simulink model "ASM_Traffic_MultiCore"  (R2026a)
settings: Solver=ode1  StartTime=SIM.tstart.v  StopTime=SIM.tend.v  FixedStep=SIM.StepSize.v
PostLoadFcn:
  | if any(exist('dsrtsu_mdlpostloadfcn', 'file') ~= 0), dsrtsu_mdlpostloadfcn('Execute', bdroot); end
  | try, asm_mdl_postloadfcn(bdroot, 'UpdateModel', 3600); catch, disp(lasterr); end,
InitFcn:
  | , if any(exist('rtifpga_mdlclblib', 'file') ~= 0), rtifpga_mdlclblib('Init', bdroot); end,
  | , if any(exist('dsmpb_private', 'file') ~= 0), dsmpb_private('dsmpb_mdlclblib', 'Init', bdroot); end,
model workspace (MAT data in the model file):
  asmReferencePath = [0 0.01 0.02 0.03 0.04 0.05 0.06 0.07 0.08 0.09 0.1 0.11 ... (350007 elements, 50001x7)]
  roadBounds : Simulink.Parameter (value not decoded)
  safetyAxes : Simulink.Parameter (value not decoded)
undefined symbols (not defined in the file): _to_, a0b2, ASM_BrakeHydraulics_DemoSystems, ASM_VehicleDynamics_DemoSystems, b98103fe8ad365046cd0, BrakeCircuit, controllerConfig, CPT, Crankshaft, DiscIntNeverNeededParam, dsmsi, FinalDriveAssembly, MDL, ModeSignals, mu, Pos_BrakePedal_Maneuver, rad, RefSignals, roadFamilyData, roadFamilyId, s_to_rpm, SIM, SoftECU, Suspension, Tire, Transmission
libraries: ASM_Traffic_lib x135, simulink x98, ASM_Utils_lib x77, ASM_VehicleDynamics_lib x70, ASM_Environment_lib x22, dsmpblib x20, dsmsilib x15, MDLD_Utils_lib x10, ASM_BrakeHydraulics_lib x3, sl_discontinuities x2
(part 22 of 65)

== system ASM_Traffic_MultiCore/Driver/Plant/UserInterface/ASMSignalBus_Plant ==
  In : Inport
  Terminator_1 : Terminator
  tag scope: ASMBUS_Driver_Plant=global
  wires:
  [ASMBUS_Driver_Plant] -> Terminator_1/1
  In/1 -> [ASMBUS_Driver_Plant]  "Plant"

== system ASM_Traffic_MultiCore/Driver/Plant/UserInterface/DISP_Plant ==
  Interface_In : Inport
  In : Inport  Port=2
  Angle_SteeringWheel[deg] : Subsystem
      mask Display: disp('')
  Bus Selector1 : BusSelector  OutputSignals=ReferenceVelocity.SpeedProfiler.a_x_Ref[m|s2],OutputSignals.Angle_SteeringWheel[deg],LateralController.PositionError.e_Lat[m]
  Bus Selector2 : BusSelector  OutputSignals=ReferenceVelocity.SpeedProfiler.v_x_Ref[km|h]
  Bus Selector3 : BusSelector  OutputSignals=OutputSignals.Pos_AccPedal[%],OutputSignals.Pos_BrakePedal[%],OutputSignals.Pos_ClutchPedal[%],OutputSignals.Gear[],OutputSignals.SelectorLever[-3T|-2P|-1R|0N|1D]
  Bus Selector4 : BusSelector  OutputSignals=ExternalModel.v_x_Vehicle[km|h]
  DRIVER : Scope  NumInputPorts=8
      settings: TimeSpan=5  ActiveDisplayYMinimum=-11.79033  ActiveDisplayYMaximum=105.56964  DataLoggingMaxPoints=20000  DataLoggingDecimation=10  DataLoggingVariableName=ScopeData2
  Err : Subsystem
  Gear[] : Subsystem
      mask Display: disp('')
  Mux : Mux  Inputs=2
  Mux1 : Mux  Inputs=3
  Mux2 : Mux  Inputs=2
  Pos_AccPedal[%] : Subsystem
      mask Display: disp('')
  Pos_BrakePedal[%] : Subsystem
      mask Display: disp('')
  Pos_ClutchPedal[%] : Subsystem
      mask Display: disp('')
  RelativeErr : Subsystem  mask{UpLim=100, LowLim=-100}
      mask prompts: UpLim "Upper Limit"; LowLim "Lower Limit"
  SelectorLever[-3T|-2P|-1R|0N|1D] : Subsystem
      mask Display: disp('')
  a_x_Vehicle_Ref[m|s2] : Subsystem
      mask Display: disp('')
  e_Lat[m] : Subsystem
      mask Display: disp('')
  v_Vehicle[km|h] : Subsystem
      mask Display: disp('')
  v_Vehicle_Ref[km|h] : Subsystem
      mask Display: disp('')
  wires:
  Angle_SteeringWheel[deg]/1(Out1) -> DRIVER/7  "Angle_SteeringWheel[deg]"
  e_Lat[m]/1(Out1) -> DRIVER/8  "e_Lat[m]"
  Bus Selector1/2 -> Angle_SteeringWheel[deg]/1(In1)  "<Angle_SteeringWheel[deg]>"
  Bus Selector1/3 -> e_Lat[m]/1(In1)  "<e_Lat[m]>"
  Bus Selector1/1 -> a_x_Vehicle_Ref[m|s2]/1(In1)  "<a_x_Ref[m|s2]>"
  a_x_Vehicle_Ref[m|s2]/1(Out1) -> DRIVER/6  "a_x_Vehicle_Ref[m|s2]"
  Bus Selector2/1 -> v_Vehicle_Ref[km|h]/1(In1)  "<v_x_Ref[km|h]>"
  In/1 -> Bus Selector3/1, Bus Selector1/1, Bus Selector2/1
  Interface_In/1 -> Bus Selector4/1
  Pos_AccPedal[%]/1(Out1) -> Mux1/1  "Pos_AccPedal[%]"
  Bus Selector3/5 -> SelectorLever[-3T|-2P|-1R|0N|1D]/1(In1)  "<SelectorLever[-3T|-2P|-1R|0N|1D]>"
  Bus Selector3/2 -> Pos_BrakePedal[%]/1(In1)  "<Pos_BrakePedal[%]>"
  Pos_BrakePedal[%]/1(Out1) -> Mux1/2  "Pos_BrakePedal[%]"
  v_Vehicle_Ref[km|h]/1(Out1) -> Err/2(Set), RelativeErr/2(Set), Mux/2
  Bus Selector3/1 -> Pos_AccPedal[%]/1(In1)  "<Pos_AccPedal[%]>"
  Mux/1 -> DRIVER/1
  Mux2/1 -> DRIVER/5
  Bus Selector3/4 -> Gear[]/1(In1)  "<Gear[]>"
  SelectorLever[-3T|-2P|-1R|0N|1D]/1(Out1) -> Mux2/2  "SelectorLever[-3T|-2P|-1R|0N|1D]"
  Pos_ClutchPedal[%]/1(Out1) -> Mux1/3  "Pos_ClutchPedal[%]"
  v_Vehicle[km|h]/1(Out1) -> Err/1(Current), RelativeErr/1(Current), Mux/1
  Bus Selector3/3 -> Pos_ClutchPedal[%]/1(In1)  "<Pos_ClutchPedal[%]>"
  Mux1/1 -> DRIVER/4
  Bus Selector4/1 -> v_Vehicle[km|h]/1(In1)  "<v_x_Vehicle[km|h]>"
  Gear[]/1(Out1) -> Mux2/1  "Gear[]"
  Err/1(Error[km|h]) -> DRIVER/3  "Error[km|h]"
  RelativeErr/1(RelativeError[%]) -> DRIVER/2  "RelativeError[%]"

== system ASM_Traffic_MultiCore/Driver/Plant/UserInterface/PAR_Plant ==
  Constant : Constant
  Out : Outport  VectorParamsAs1DForOutWhenUnconnected=off
  wires:
  Constant/1 -> Out/1

== system ASM_Traffic_MultiCore/Driver/SignalInterface/ASMSignalInterface/signal_structure ==
  ASMSignalBus : Inport
  BusSelector_1 : BusSelector  OutputSignals=LongitudinalController,LateralController,ReferenceVelocity,OutputSignals
  ContentID : Constant  Value=913375857
  Curvature : BusSelector  OutputSignals=Curv_Vehicle[1|m],Curv_Preview[1|m]
  GearShifter : BusSelector  OutputSignals=Pos_AccPedal[%],Pos_BrakePedal[%],Pos_ClutchPedal[%],Gear[],SelectorLever[-3T|-2P|-1R|0N|1D]
  InfoBlock : Subsystem
      mask Display: fprintf('Structural changes of the signal bus require an update \nof the ''ASMSignalCollector'' block. \n\nTo start the update process double click the parent block.\n\n WARNING:\n During update this subsystem will be cleared completely')
  LatCtrl1 : BusSelector  OutputSignals=s_Preview_Lat[m],Angle_Steering[rad],Angle_SteeringWheel[deg]
  LatCtrl2 : BusSelector  OutputSignals=Angle_SteeringWheel[deg],Angle_Steering[deg],s_Preview_Lat[m],e_Yaw[deg],e_Lat[m],e_Lat_Preview[m]
  LateralController : BusSelector  OutputSignals=LatCtrl1,LatCtrl2,PositionError
  LongCtrl : BusSelector  OutputSignals=t_Preview[s],Pos_AccPedal[%],Pos_BrakePedal[%]
  LongitudinalController : BusSelector  OutputSignals=LongCtrl,GearShifter
  MDLD_DATA_CAPTURE : MDLD_Utils_lib/ModelDeskPlotInterface/DataCapture_Sfcn/MDLD_DATA_CAPTURE  inputPortWidth=100  measurementSignals=[0 0 0 0 0 0 0 0 0 0 0 0 0 0 0 0 0 0 0 0 0 0 0 0 0 0 0 0 0 0 0 0 0 0 0 0 0 0 0 0 0 0 0 0 0 0 0 0 0 0 0 0 0 0 0 0 0 0 0 0 0 0 0 0 0 0 0 0 0 0 0 0 0 0 0 0 0 0 0 0 0 0 0 0 0 0 0 0 0 0 0 0 0 0 0 0 0 0 0 0]  downsampling=1  samplingPeriod=SIM.StepSize.v  uuid=0  ASMProperties=struct('Name','mdld_data_capture','Version','1.0','Library','mdld_utils_lib')  startTriggerDelay=0  startTriggerLogic=0  startTriggerCount=0  startTriggerConditions=[0,0,0,0,0,0,0,0,0]  stopTriggerDelay=0  stopTriggerLogic=0  stopTriggerCount=0  stopTriggerConditions=[0,0,0,0,0,0,0,0,0]  ContentID_RefStruct=913375857
  OutputSignals : BusSelector  OutputSignals=Pos_AccPedal[%],Pos_BrakePedal[%],Pos_ClutchPedal[%],Gear[],SelectorLever[-3T|-2P|-1R|0N|1D],s_Preview_vRef[m],s_Preview_LatCtrl[m],s_Preview[m],Angle_SteeringWheel[deg]
  PositionError : BusSelector  OutputSignals=e_Lat[m],e_Lat_Abs[m],e_Total[m]
  ReferenceVelocity : BusSelector  OutputSignals=SpeedProfiler,Curvature
  Reshape_{17,29,35..37} (5 alike) : Reshape
  SignalFilter : Mux  Inputs=38
  SignalFilterGain : Gain
  SpeedProfiler : BusSelector  OutputSignals=v_x_Ref[m|s],v_x_Ref[km|h],v_x_Ref_Preview[m|s],v_x_Ref_Preview[km|h],a_x_Ref[m|s2],a_y_Ref[m|s2],s_Preview_vRef[m]
  Terminator : Terminator
  wires:
  ASMSignalBus/1 -> BusSelector_1/1
  BusSelector_1/1 -> LongitudinalController/1  "<LongitudinalController>"
  LongitudinalController/1 -> LongCtrl/1  "<LongCtrl>"
  LongitudinalController/2 -> GearShifter/1  "<GearShifter>"
  BusSelector_1/2 -> LateralController/1  "<LateralController>"
  LateralController/1 -> LatCtrl1/1  "<LatCtrl1>"
  LateralController/2 -> LatCtrl2/1  "<LatCtrl2>"
  LateralController/3 -> PositionError/1  "<PositionError>"
  BusSelector_1/3 -> ReferenceVelocity/1  "<ReferenceVelocity>"
  ReferenceVelocity/1 -> SpeedProfiler/1  "<SpeedProfiler>"
  ReferenceVelocity/2 -> Curvature/1  "<Curvature>"
  BusSelector_1/4 -> OutputSignals/1  "<OutputSignals>"
  ContentID/1 -> Terminator/1
  LongCtrl/1 -> SignalFilter/1  "<t_Preview[s]>"
  LongCtrl/2 -> SignalFilter/2  "<Pos_AccPedal[%]>"
  LongCtrl/3 -> SignalFilter/3  "<Pos_BrakePedal[%]>"
  GearShifter/1 -> SignalFilter/4  "<Pos_AccPedal[%]>"
  GearShifter/2 -> SignalFilter/5  "<Pos_BrakePedal[%]>"
  GearShifter/3 -> SignalFilter/6  "<Pos_ClutchPedal[%]>"
  GearShifter/4 -> SignalFilter/7  "<Gear[]>"
  GearShifter/5 -> SignalFilter/8  "<SelectorLever[-3T|-2P|-1R|0N|1D]>"
  LatCtrl1/1 -> SignalFilter/9  "<s_Preview_Lat[m]>"
  LatCtrl1/2 -> SignalFilter/10  "<Angle_Steering[rad]>"
  LatCtrl1/3 -> SignalFilter/11  "<Angle_SteeringWheel[deg]>"
  LatCtrl2/1 -> SignalFilter/12  "<Angle_SteeringWheel[deg]>"
  LatCtrl2/2 -> SignalFilter/13  "<Angle_Steering[deg]>"
  LatCtrl2/3 -> SignalFilter/14  "<s_Preview_Lat[m]>"
  LatCtrl2/4 -> SignalFilter/15  "<e_Yaw[deg]>"
  LatCtrl2/5 -> SignalFilter/16  "<e_Lat[m]>"
  LatCtrl2/6 -> Reshape_17/1  "<e_Lat_Preview[m]>"
  Reshape_17/1 -> SignalFilter/17
  PositionError/1 -> SignalFilter/18  "<e_Lat[m]>"
  PositionError/2 -> SignalFilter/19  "<e_Lat_Abs[m]>"
  PositionError/3 -> SignalFilter/20  "<e_Total[m]>"
  SpeedProfiler/1 -> SignalFilter/21  "<v_x_Ref[m|s]>"
  SpeedProfiler/2 -> SignalFilter/22  "<v_x_Ref[km|h]>"
  SpeedProfiler/3 -> SignalFilter/23  "<v_x_Ref_Preview[m|s]>"
  SpeedProfiler/4 -> SignalFilter/24  "<v_x_Ref_Preview[km|h]>"
  SpeedProfiler/5 -> SignalFilter/25  "<a_x_Ref[m|s2]>"
  SpeedProfiler/6 -> SignalFilter/26  "<a_y_Ref[m|s2]>"
  SpeedProfiler/7 -> SignalFilter/27  "<s_Preview_vRef[m]>"
  Curvature/1 -> SignalFilter/28  "<Curv_Vehicle[1|m]>"
  Curvature/2 -> Reshape_29/1  "<Curv_Preview[1|m]>"
  Reshape_29/1 -> SignalFilter/29
  OutputSignals/1 -> SignalFilter/30  "<Pos_AccPedal[%]>"
  OutputSignals/2 -> SignalFilter/31  "<Pos_BrakePedal[%]>"
  OutputSignals/3 -> SignalFilter/32  "<Pos_ClutchPedal[%]>"
  OutputSignals/4 -> SignalFilter/33  "<Gear[]>"
  OutputSignals/5 -> SignalFilter/34  "<SelectorLever[-3T|-2P|-1R|0N|1D]>"
  OutputSignals/6 -> Reshape_35/1  "<s_Preview_vRef[m]>"
  Reshape_35/1 -> SignalFilter/35
  OutputSignals/7 -> Reshape_36/1  "<s_Preview_LatCtrl[m]>"
  Reshape_36/1 -> SignalFilter/36
  OutputSignals/8 -> Reshape_37/1  "<s_Preview[m]>"
  Reshape_37/1 -> SignalFilter/37
  OutputSignals/9 -> SignalFilter/38  "<Angle_SteeringWheel[deg]>"
  SignalFilter/1 -> SignalFilterGain/1
  SignalFilterGain/1 -> MDLD_DATA_CAPTURE/1

== system ASM_Traffic_MultiCore/Driver/SignalInterface/ExternalOutports/Select_Outport_Signals ==
  ASMSignalBus : Inport
  Bus Selector : BusSelector  OutputSignals=OutputSignals.Pos_AccPedal[%],OutputSignals.Pos_BrakePedal[%],OutputSignals.Pos_ClutchPedal[%],OutputSignals.Gear[],OutputSignals.SelectorLever[-3T|-2P|-1R|0N|1D],OutputSignals.Angle_SteeringWheel[deg],ReferenceVelocity.SpeedProfiler.v_x_Ref[km|h],ReferenceVelocity.SpeedProfiler.a_x_Ref[m|s2],ReferenceVelocity.SpeedProfiler.a_y_Ref[m|s2]
  Pos_AccPedal[%] : Outport  VectorParamsAs1DForOutWhenUnconnected=off
  Pos_BrakePedal[%] : Outport  Port=2  VectorParamsAs1DForOutWhenUnconnected=off
  Pos_ClutchPedal[%] : Outport  Port=3  VectorParamsAs1DForOutWhenUnconnected=off
  Gear[] : Outport  Port=4  VectorParamsAs1DForOutWhenUnconnected=off
  SelectorLever[-3T|-2P|-1R|0N|1D] : Outport  Port=5  VectorParamsAs1DForOutWhenUnconnected=off
  Angle_SteeringWheel[deg] : Outport  Port=6  VectorParamsAs1DForOutWhenUnconnected=off
  v_x_Ref[km|h] : Outport  Port=7  VectorParamsAs1DForOutWhenUnconnected=off
  a_x_Ref[m|s2] : Outport  Port=8  VectorParamsAs1DForOutWhenUnconnected=off
  a_y_Ref[m|s2] : Outport  Port=9  VectorParamsAs1DForOutWhenUnconnected=off
  wires:
  ASMSignalBus/1 -> Bus Selector/1
  Bus Selector/1 -> Pos_AccPedal[%]/1  "<Pos_AccPedal[%]>"
  Bus Selector/2 -> Pos_BrakePedal[%]/1  "<Pos_BrakePedal[%]>"
  Bus Selector/3 -> Pos_ClutchPedal[%]/1  "<Pos_ClutchPedal[%]>"
  Bus Selector/4 -> Gear[]/1  "<Gear[]>"
  Bus Selector/5 -> SelectorLever[-3T|-2P|-1R|0N|1D]/1  "<SelectorLever[-3T|-2P|-1R|0N|1D]>"
  Bus Selector/6 -> Angle_SteeringWheel[deg]/1  "<Angle_SteeringWheel[deg]>"
  Bus Selector/7 -> v_x_Ref[km|h]/1  "<v_x_Ref[km|h]>"
  Bus Selector/8 -> a_x_Ref[m|s2]/1  "<a_x_Ref[m|s2]>"
  Bus Selector/9 -> a_y_Ref[m|s2]/1  "<a_y_Ref[m|s2]>"

== system ASM_Traffic_MultiCore/Drivetrain/Control/SoftECU_Drivetrain/SoftECU_Transmission ==
  n_Engine[rad|s] : Inport  PortDimensions=1
  omega_In_Trm[rad|s] : Inport  Port=2  PortDimensions=1
  omega_Out_Trm[rad|s] : Inport  Port=3
  Gear_Current[] : Inport  Port=4
  Pos_AccPedal_Driver[%] : Inport  Port=5
  SelectorLever[-3T|-2P|-1R|0N|1D] : Inport  Port=6  PortDimensions=1
  TipShift[-1Down|0Off|1Up] : Inport  Port=7
  Gear_Max_Maneuver[0Off|1_n] : Inport  Port=8
  Reset[0|1] : Inport  Port=9
  Gear_Maneuver[] : Inport  Port=10
  GearClutch_Mode[1Stim|2SoftECU|3OpenClutch|4RefGear] : Inport  Port=11
  State_Engine[0|1|2|3|4] : Inport  Port=12
  State_StartStop[1Off|2NotReady|3Ready|4EngStopped] : Inport  Port=13
  Enable_v_Init[0|1] : Inport  Port=14
  ASMSignalCollector : Subsystem
  Ctrl_Lockup_Clutch_Maneuver[0_1] : Constant  Value=0
  Gear_Requested : Sum  SaturateOnIntegerOverflow=on
  Goto Tag Visibility5 : GotoTagVisibility  GotoTag=TAG_SoftECU_Const_Max_num_Gear
  Goto Tag Visibility : GotoTagVisibility  GotoTag=ASMBUS_SOFTECU_LOCKUP_CLUTCH_CONTROL
  Goto Tag Visibility1 : GotoTagVisibility  GotoTag=ASMBUS_SOFTECU_SHIFT_STRATEGY
  Goto Tag Visibility2 : GotoTagVisibility  GotoTag=ASMBUS_SOFTECU_TIP_SHIFT_CONTROL
  Goto Tag Visibility3 : GotoTagVisibility  GotoTag=ASMBUS_SOFTECU_TORQUE_INTERVENTION_CONTROL
  Goto Tag Visibility4 : GotoTagVisibility  GotoTag=ASMBUS_SOFTECU_SHIFT_LOCK_CONTROL
  LOCKUP_CLUTCH_CONTROL : ASM_VehicleDynamics_lib/SoftECU/SoftECU_Transmission/LOCKUP_CLUTCH_CONTROL  Tag=ASM_SUBCOMPONENT  Const_P_LockupClutch=MDL.SoftECU.SoftECUTransmission.LockupClutchControl.Const_P_LockupClutch  Const_I_LockupClutch=MDL.SoftECU.SoftECUTransmission.LockupClutchControl.Const_I_LockupClutch  Map_State_LockupClutch=MDL.SoftECU.SoftECUTransmission.LockupClutchControl.Map_State_LockupClutch  StepSize=SIM.StepSize  ASMProperties=struct('Name','LOCKUP_CLUTCH_CONTROL','Version','2.0','Library','ASM_VehicleDynamics_lib')  ASMInstanceName=lockup_clutch_control  ASMInstanceID=1
  Memory : Memory
  Memory1 : Memory  InitialCondition=100
  SHIFT_LOCK_CONTROL : ASM_VehicleDynamics_lib/SoftECU/SoftECU_Transmission/SHIFT_LOCK_CONTROL  Tag=ASM_SUBCOMPONENT  ASMProperties=struct('Name','SHIFT_LOCK_CONTROL','Version','2.0','Library','ASM_VehicleDynamics_lib')  ASMInstanceName=shift_lock_control  ASMInstanceID=1
  SHIFT_STRATEGY : ASM_VehicleDynamics_lib/SoftECU/SoftECU_Transmission/SHIFT_STRATEGY  Tag=ASM_SUBCOMPONENT  Map_omega_Upshift=MDL.SoftECU.SoftECUTransmission.ShiftStrategy.Map_omega_Upshift  Map_omega_Downshift=MDL.SoftECU.SoftECUTransmission.ShiftStrategy.Map_omega_Downshift  Const_t_Min_Shift=MDL.SoftECU.SoftECUTransmission.ShiftStrategy.Const_t_Min_Shift  StepSize=SIM.StepSize  ASMProperties=struct('Name','SHIFT_STRATEGY','Version','2.0','Library','ASM_VehicleDynamics_lib')  ASMInstanceName=shift_strategy  ASMInstanceID=1
  SOFTECU_SETUP : Subsystem
  State_Engine : Subsystem
      mask Display: fprintf('Engine State')
  Sw_Gear : Subsystem
  Sw_LockupClutch : Subsystem
  TIP_SHIFT_CONTROL : ASM_VehicleDynamics_lib/SoftECU/SoftECU_Transmission/TIP_SHIFT_CONTROL  Tag=ASM_SUBCOMPONENT  ASMProperties=struct('Name','TIP_SHIFT_CONTROL','Version','1.0','Library','ASM_VehicleDynamics_lib')  ASMInstanceName=tip_shift_control  ASMInstanceID=1
  TORQUE_INTERVENTION_CONTROL : ASM_VehicleDynamics_lib/SoftECU/SoftECU_Transmission/TORQUE_INTERVENTION_CONTROL  Tag=ASM_SUBCOMPONENT  Map_Factor_Trq_Engine_Red=MDL.SoftECU.SoftECUTransmission.TorqueInterventionControl.Map_Factor_Trq_Engine_Red  Const_t_Gear_Offs=MDL.SoftECU.SoftECUTransmission.TorqueInterventionControl.Const_t_Gear_Offs  StepSize=SIM.StepSize  ASMProperties=struct('Name','TORQUE_INTERVENTION_CONTROL','Version','3.0','Library','ASM_VehicleDynamics_lib')  ASMInstanceName=torque_intervention_control  ASMInstanceID=1
  Unit Delay : Subsystem
  Unit Delay2 : Subsystem
  UnitConversion1 : ASM_Utils_lib/UnitConversion/UnitConversion  Selection=rad/s_to_rpm
  UnitConversion2 : ASM_Utils_lib/UnitConversion/UnitConversion  Selection=rad/s_to_rpm
  UnitConversion3 : ASM_Utils_lib/UnitConversion/UnitConversion  Selection=rad/s_to_rpm
  ASMSignalBus : Outport  VectorParamsAs1DForOutWhenUnconnected=off
  Factor_Trq_Engine_Red[%] : Outport  Port=2  VectorParamsAs1DForOutWhenUnconnected=off
  Ctrl_Parking_Pawl[0|1] : Outport  Port=3  VectorParamsAs1DForOutWhenUnconnected=off
  Ctrl_Lockup_Clutch[0_1] : Outport  Port=4  VectorParamsAs1DForOutWhenUnconnected=off
  Gear[] : Outport  Port=5  VectorParamsAs1DForOutWhenUnconnected=off
  tag scope: ASMBUS_SOFTECU_LOCKUP_CLUTCH_CONTROL=scoped, ASMBUS_SOFTECU_SHIFT_LOCK_CONTROL=scoped, ASMBUS_SOFTECU_SHIFT_STRATEGY=scoped, ASMBUS_SOFTECU_TIP_SHIFT_CONTROL=scoped, ASMBUS_SOFTECU_TORQUE_INTERVENTION_CONTROL=scoped
  wires:
  Memory1/1 -> Factor_Trq_Engine_Red[%]/1
  Reset[0|1]/1 -> LOCKUP_CLUTCH_CONTROL/7, Unit Delay2/2(Reset_States[0|1]), Unit Delay/2(Reset_States[0|1]), TORQUE_INTERVENTION_CONTROL/2, TIP_SHIFT_CONTROL/5, SHIFT_STRATEGY/7, SHIFT_LOCK_CONTROL/2
  State_StartStop[1Off|2NotReady|3Ready|4EngStopped]/1 -> State_Engine/2(State_StartStop[1Off|2NotReady|3Ready|4EngStopped])
  State_Engine/1(Out[]) -> SHIFT_STRATEGY/6, TIP_SHIFT_CONTROL/4
  ASMSignalCollector/1(ASMSignalBus) -> ASMSignalBus/1
  TIP_SHIFT_CONTROL/1 -> [ASMBUS_SOFTECU_TIP_SHIFT_CONTROL]
  SHIFT_STRATEGY/1 -> [ASMBUS_SOFTECU_SHIFT_STRATEGY]
  LOCKUP_CLUTCH_CONTROL/1 -> [ASMBUS_SOFTECU_LOCKUP_CLUTCH_CONTROL]
  UnitConversion1/1 -> LOCKUP_CLUTCH_CONTROL/2
  omega_In_Trm[rad|s]/1 -> UnitConversion1/1
  UnitConversion3/1 -> LOCKUP_CLUTCH_CONTROL/1
  n_Engine[rad|s]/1 -> UnitConversion3/1
  Ctrl_Lockup_Clutch_Maneuver[0_1]/1 -> LOCKUP_CLUTCH_CONTROL/3
  TipShift[-1Down|0Off|1Up]/1 -> TIP_SHIFT_CONTROL/3
  Gear_Current[]/1 -> TIP_SHIFT_CONTROL/2
  omega_Out_Trm[rad|s]/1 -> UnitConversion2/1
  Gear_Maneuver[]/1 -> SHIFT_STRATEGY/3
  GearClutch_Mode[1Stim|2SoftECU|3OpenClutch|4RefGear]/1 -> Sw_LockupClutch/1(In[]), Sw_Gear/1(In[])
  SelectorLever[-3T|-2P|-1R|0N|1D]/1 -> SHIFT_LOCK_CONTROL/1, TIP_SHIFT_CONTROL/1, SHIFT_STRATEGY/1
  Gear_Max_Maneuver[0Off|1_n]/1 -> SOFTECU_SETUP/1(Gear_Max_Maneuver[0Off|1_n])
  Unit Delay2/1(Out1) -> Ctrl_Lockup_Clutch[0_1]/1
  Memory/1 -> Gear[]/1
  Unit Delay/1(Out1) -> Ctrl_Parking_Pawl[0|1]/1
  SHIFT_LOCK_CONTROL/2 -> Unit Delay/1(In1)
  LOCKUP_CLUTCH_CONTROL/2 -> Unit Delay2/1(In1)
  TIP_SHIFT_CONTROL/2 -> Gear_Requested/2
  SHIFT_STRATEGY/2 -> Gear_Requested/1
  Gear_Requested/1 -> TORQUE_INTERVENTION_CONTROL/1
  UnitConversion2/1 -> LOCKUP_CLUTCH_CONTROL/4, SHIFT_STRATEGY/2
  State_Engine[0|1|2|3|4]/1 -> State_Engine/1(In[])
  Sw_LockupClutch/1(Out[]) -> LOCKUP_CLUTCH_CONTROL/5
  Sw_Gear/1(Out[]) -> SHIFT_STRATEGY/4
  SHIFT_LOCK_CONTROL/1 -> [ASMBUS_SOFTECU_SHIFT_LOCK_CONTROL]
  Pos_AccPedal_Driver[%]/1 -> LOCKUP_CLUTCH_CONTROL/6, SHIFT_STRATEGY/5
  TORQUE_INTERVENTION_CONTROL/1 -> [ASMBUS_SOFTECU_TORQUE_INTERVENTION_CONTROL]
  TORQUE_INTERVENTION_CONTROL/3 -> Memory/1
  TORQUE_INTERVENTION_CONTROL/2 -> Memory1/1
  Enable_v_Init[0|1]/1 -> TORQUE_INTERVENTION_CONTROL/3, SHIFT_STRATEGY/8

== system ASM_Traffic_MultiCore/Drivetrain/Control/Sw_ECU_Signals/Ctrl_CentralDiff[0_1] ==
  SoftECU : Inport
  RealECU : Inport  Port=2
  Const_Ctrl_CentralDiff[0_1] : Constant  Value=0
  MultiPortSwitch : MultiPortSwitch
  Sw_Ctrl_CentralDiff[1SoftECU|2RealECU|3Const] : Constant  Value=CPT.MDL_SW.Sw_Ctrl_CentralDiff.v
  Ctrl_CentralDiff[0_1] : Outport  VectorParamsAs1DForOutWhenUnconnected=off
  wires:
  Sw_Ctrl_CentralDiff[1SoftECU|2RealECU|3Const]/1 -> MultiPortSwitch/1
  SoftECU/1 -> MultiPortSwitch/2
  RealECU/1 -> MultiPortSwitch/3
  Const_Ctrl_CentralDiff[0_1]/1 -> MultiPortSwitch/4
  MultiPortSwitch/1 -> Ctrl_CentralDiff[0_1]/1

== system ASM_Traffic_MultiCore/Drivetrain/Control/Sw_ECU_Signals/Ctrl_Clutch_4WD[0_1] ==
  SoftECU : Inport
  RealECU : Inport  Port=2
  Const_Ctrl_Clutch_4WD[0_1] : Constant  Value=0
  MultiPortSwitch : MultiPortSwitch
  Sw_Clutch_4WD[1SoftECU|2RealECU|3Const] : Constant  Value=CPT.MDL_SW.Sw_Clutch_4WD.v
  Ctrl_Clutch_4WD[0_1] : Outport  VectorParamsAs1DForOutWhenUnconnected=off
  wires:
  Sw_Clutch_4WD[1SoftECU|2RealECU|3Const]/1 -> MultiPortSwitch/1
  SoftECU/1 -> MultiPortSwitch/2
  RealECU/1 -> MultiPortSwitch/3
  Const_Ctrl_Clutch_4WD[0_1]/1 -> MultiPortSwitch/4
  MultiPortSwitch/1 -> Ctrl_Clutch_4WD[0_1]/1

== system ASM_Traffic_MultiCore/Drivetrain/Control/Sw_ECU_Signals/Ctrl_FrontDiff[0_1] ==
  SoftECU : Inport
  RealECU : Inport  Port=2
  Const_Ctrl_FrontDiff[0_1] : Constant  Value=0
  MultiPortSwitch : MultiPortSwitch
  Sw_Ctrl_FrontDiff[1SoftECU|2RealECU|3Const] : Constant  Value=CPT.MDL_SW.Sw_Ctrl_FrontDiff.v
  Ctrl_FrontDiff[0_1] : Outport  VectorParamsAs1DForOutWhenUnconnected=off
  wires:
  MultiPortSwitch/1 -> Ctrl_FrontDiff[0_1]/1
  Const_Ctrl_FrontDiff[0_1]/1 -> MultiPortSwitch/4
  RealECU/1 -> MultiPortSwitch/3
  SoftECU/1 -> MultiPortSwitch/2
  Sw_Ctrl_FrontDiff[1SoftECU|2RealECU|3Const]/1 -> MultiPortSwitch/1

== system ASM_Traffic_MultiCore/Drivetrain/Control/Sw_ECU_Signals/Ctrl_Lockup_Clutch[0_1] ==
  SoftECU : Inport
  RealECU : Inport  Port=2
  Const_Ctrl_Lockup_Clutch[0_1] : Constant  Value=0
  MultiPortSwitch : MultiPortSwitch
  Sw_Ctrl_Lockup_Clutch[1SoftECU|2RealECU|3Const] : Constant  Value=CPT.MDL_SW.Sw_Ctrl_Lockup_Clutch.v
  Ctrl_Lockup_Clutch[0_1] : Outport  VectorParamsAs1DForOutWhenUnconnected=off
  wires:
  MultiPortSwitch/1 -> Ctrl_Lockup_Clutch[0_1]/1
  Const_Ctrl_Lockup_Clutch[0_1]/1 -> MultiPortSwitch/4
  RealECU/1 -> MultiPortSwitch/3
  SoftECU/1 -> MultiPortSwitch/2
  Sw_Ctrl_Lockup_Clutch[1SoftECU|2RealECU|3Const]/1 -> MultiPortSwitch/1

== system ASM_Traffic_MultiCore/Drivetrain/Control/Sw_ECU_Signals/Ctrl_Parking_Pawl[0|1] ==
  SoftECU : Inport
  RealECU : Inport  Port=2
  Const_Park_Lock[0|1] : Constant  Value=0
  MultiPortSwitch : MultiPortSwitch
  Sw_Parking_Pawl[1SoftECU|2RealECU|3Const] : Constant  Value=CPT.MDL_SW.Sw_Parking_Pawl.v
  Ctrl_Parking_Pawl[0|1] : Outport  VectorParamsAs1DForOutWhenUnconnected=off
  wires:
  MultiPortSwitch/1 -> Ctrl_Parking_Pawl[0|1]/1
  Const_Park_Lock[0|1]/1 -> MultiPortSwitch/4
  RealECU/1 -> MultiPortSwitch/3
  SoftECU/1 -> MultiPortSwitch/2
  Sw_Parking_Pawl[1SoftECU|2RealECU|3Const]/1 -> MultiPortSwitch/1

== system ASM_Traffic_MultiCore/Drivetrain/Control/Sw_ECU_Signals/Ctrl_RearDiff[0_1] ==
  SoftECU : Inport
  RealECU : Inport  Port=2
  Const_Ctrl_RearDiff[0_1] : Constant  Value=0
  MultiPortSwitch : MultiPortSwitch
  Sw_Ctrl_RearDiff[1SoftECU|2RealECU|3Const] : Constant  Value=CPT.MDL_SW.Sw_Ctrl_RearDiff.v
  Ctrl_RearDiff[0_1] : Outport  VectorParamsAs1DForOutWhenUnconnected=off
  wires:
  Sw_Ctrl_RearDiff[1SoftECU|2RealECU|3Const]/1 -> MultiPortSwitch/1
  SoftECU/1 -> MultiPortSwitch/2
  RealECU/1 -> MultiPortSwitch/3
  Const_Ctrl_RearDiff[0_1]/1 -> MultiPortSwitch/4
  MultiPortSwitch/1 -> Ctrl_RearDiff[0_1]/1

== system ASM_Traffic_MultiCore/Drivetrain/Control/Sw_ECU_Signals/Factor_Trq_Engine_Red[%] ==
  SoftECU : Inport
  RealECU : Inport  Port=2
  Const_Factor_Trq_Engine_Red[%] : Constant  Value=0
  MultiPortSwitch : MultiPortSwitch
  Sw_Factor_Trq_Engine_Redl[1SoftECU|2RealECU|3Const] : Constant
  Factor_Trq_Engine_Red[%] : Outport  VectorParamsAs1DForOutWhenUnconnected=off
  wires:
  Sw_Factor_Trq_Engine_Redl[1SoftECU|2RealECU|3Const]/1 -> MultiPortSwitch/1
  SoftECU/1 -> MultiPortSwitch/2
  RealECU/1 -> MultiPortSwitch/3
  Const_Factor_Trq_Engine_Red[%]/1 -> MultiPortSwitch/4
  MultiPortSwitch/1 -> Factor_Trq_Engine_Red[%]/1

== system ASM_Traffic_MultiCore/Drivetrain/Control/Sw_ECU_Signals/Gear[] ==
  SoftECU : Inport
  RealECU : Inport  Port=2
  Const_Gear[] : Constant  Value=0
  MultiPortSwitch : MultiPortSwitch
  Sw_Gear[1SoftECU|2RealECU|3Const] : Constant  Value=CPT.MDL_SW.Sw_Gear.v
  Gear[] : Outport  VectorParamsAs1DForOutWhenUnconnected=off
  wires:
  Sw_Gear[1SoftECU|2RealECU|3Const]/1 -> MultiPortSwitch/1
  SoftECU/1 -> MultiPortSwitch/2
  RealECU/1 -> MultiPortSwitch/3
  Const_Gear[]/1 -> MultiPortSwitch/4
  MultiPortSwitch/1 -> Gear[]/1

== system ASM_Traffic_MultiCore/Drivetrain/Control/UserInterface/ASMSignalBus_Control ==
  In : Inport
  Terminator_1 : Terminator
  tag scope: ASMBUS_Drivetrain_Control=global
  wires:
  In/1 -> [ASMBUS_Drivetrain_Control]  "Control"
  [ASMBUS_Drivetrain_Control] -> Terminator_1/1

== system ASM_Traffic_MultiCore/Drivetrain/Control/UserInterface/DISP_Control ==
  In : Inport
  Bus Selector1 : BusSelector  OutputSignals=Lockup_Clutch_Control.Ctrl_Lockup_Clutch[0_1],Torque_Intervention_Control.Gear[],Torque_Intervention_Control.Factor_Trq_Engine_Red[%],Shift_Lock_Control.Ctrl_Parking_Pawl[0|1]
  Ctrl_Lockup_Clutch[0_1] : Subsystem
      mask Display: disp('')
  Ctrl_Parking_Pawl[0|1] : Subsystem
      mask Display: disp('')
  Factor_Trq_Engine_Red[%] : Subsystem
      mask Display: disp('')
  Gear[] : Subsystem
      mask Display: disp('')
  SoftECUTransmission : Scope  NumInputPorts=4
      settings: TimeSpan=5  ActiveDisplayYMinimum=2  ActiveDisplayYMaximum=4  DataLoggingMaxPoints=20000  DataLoggingDecimation=10  DataLoggingVariableName=ScopeData7
  wires:
  In/1 -> Bus Selector1/1
  Bus Selector1/4 -> Ctrl_Parking_Pawl[0|1]/1(In1)  "<Ctrl_Parking_Pawl[0|1]>"
  Ctrl_Parking_Pawl[0|1]/1(Out1) -> SoftECUTransmission/4  "Ctrl_Parking_Pawl[0|1]"
  Factor_Trq_Engine_Red[%]/1(Out1) -> SoftECUTransmission/3  "Factor_Trq_Engine_Red[%]"
  Bus Selector1/3 -> Factor_Trq_Engine_Red[%]/1(In1)  "<Factor_Trq_Engine_Red[%]>"
  Bus Selector1/1 -> Ctrl_Lockup_Clutch[0_1]/1(In1)  "<Ctrl_Lockup_Clutch[0_1]>"
  Bus Selector1/2 -> Gear[]/1(In1)  "<Gear[]>"
  Gear[]/1(Out1) -> SoftECUTransmission/2  "Gear[]"
  Ctrl_Lockup_Clutch[0_1]/1(Out1) -> SoftECUTransmission/1  "Ctrl_Lockup_Clutch[0_1]"

== system ASM_Traffic_MultiCore/Drivetrain/Control/UserInterface/PAR_Control ==
  Constant : Constant  Value=0
  Out : Outport  VectorParamsAs1DForOutWhenUnconnected=off
  wires:
  Constant/1 -> Out/1

== system ASM_Traffic_MultiCore/Drivetrain/Interface_In/ExternalSignals/ExternalECU_Transmission ==
  Factor_Trq_Engine_Red[%] : Inport
  Ctrl_Parking_Pawl[0|1] : Inport  Port=2
  Ctrl_Lockup_Clutch[0_1] : Inport  Port=3
  Gear[] : Inport  Port=4
  Ctrl_CentralDiff[0_1] : Inport  Port=5
  Ctrl_FrontDiff[0_1] : Inport  Port=6
  Ctrl_RearDiff[0_1] : Inport  Port=7
  Ctrl_Clutch_4WD[0_1] : Inport  Port=8
  Bus Creator : BusCreator  Inputs=8
  Out : Outport  VectorParamsAs1DForOutWhenUnconnected=off
  wires:
  Bus Creator/1 -> Out/1  "ExternalECU"
  Gear[]/1 -> Bus Creator/4  "Gear[]"
  Ctrl_Lockup_Clutch[0_1]/1 -> Bus Creator/3  "Ctrl_Lockup_Clutch[0_1]"
  Ctrl_Parking_Pawl[0|1]/1 -> Bus Creator/2  "Ctrl_Parking_Pawl[0|1]"
  Factor_Trq_Engine_Red[%]/1 -> Bus Creator/1  "Factor_Trq_Engine_Red[%]"
  Ctrl_CentralDiff[0_1]/1 -> Bus Creator/5  "Ctrl_CentralDiff[0_1]"
  Ctrl_FrontDiff[0_1]/1 -> Bus Creator/6  "Ctrl_FrontDiff[0_1]"
  Ctrl_RearDiff[0_1]/1 -> Bus Creator/7  "Ctrl_RearDiff[0_1]"
  Ctrl_Clutch_4WD[0_1]/1 -> Bus Creator/8  "Ctrl_Clutch_4WD[0_1]"

== system ASM_Traffic_MultiCore/Drivetrain/Interface_In/ModelSignals/CrankAngle_Cyl[aTDC]_ ==
  In1 : Inport
  DummyGain : Gain  SaturateOnIntegerOverflow=on  OutDataTypeStr=Inherit: Same as input  ParamDataTypeStr=Inherit: Same as input
  Out1 : Outport  VectorParamsAs1DForOutWhenUnconnected=off
  wires:
  In1/1 -> DummyGain/1
  DummyGain/1 -> Out1/1

== system ASM_Traffic_MultiCore/Drivetrain/Interface_In/ModelSignals/Enable_v_Init[0|1]_ ==
  In1 : Inport
  DummyGain : Gain  SaturateOnIntegerOverflow=on  OutDataTypeStr=Inherit: Same as input  ParamDataTypeStr=Inherit: Same as input
  Out1 : Outport  VectorParamsAs1DForOutWhenUnconnected=off
  wires:
  In1/1 -> DummyGain/1
  DummyGain/1 -> Out1/1

== system ASM_Traffic_MultiCore/Drivetrain/Interface_In/ModelSignals/Gear[]_ ==
  In1 : Inport
  DummyGain : Gain  SaturateOnIntegerOverflow=on  OutDataTypeStr=Inherit: Same as input  ParamDataTypeStr=Inherit: Same as input
  Out1 : Outport  VectorParamsAs1DForOutWhenUnconnected=off
  wires:
  In1/1 -> DummyGain/1
  DummyGain/1 -> Out1/1

== system ASM_Traffic_MultiCore/Drivetrain/Interface_In/ModelSignals/Gear_Maneuver[]_ ==
  In1 : Inport
  DummyGain : Gain  SaturateOnIntegerOverflow=on  OutDataTypeStr=Inherit: Same as input  ParamDataTypeStr=Inherit: Same as input
  Out1 : Outport  VectorParamsAs1DForOutWhenUnconnected=off
  wires:
  DummyGain/1 -> Out1/1
  In1/1 -> DummyGain/1

== system ASM_Traffic_MultiCore/Drivetrain/Interface_In/ModelSignals/Gear_Max[0Off|1_n]_ ==
  In1 : Inport
  DummyGain : Gain  SaturateOnIntegerOverflow=on  OutDataTypeStr=Inherit: Same as input  ParamDataTypeStr=Inherit: Same as input
  Out1 : Outport  VectorParamsAs1DForOutWhenUnconnected=off
  wires:
  DummyGain/1 -> Out1/1
  In1/1 -> DummyGain/1

== system ASM_Traffic_MultiCore/Drivetrain/Interface_In/ModelSignals/Mode_GearClutch[1Stim|2Driver|3OpenClutch|4RefGear]_ ==
  In1 : Inport
  DummyGain : Gain  SaturateOnIntegerOverflow=on  OutDataTypeStr=Inherit: Same as input  ParamDataTypeStr=Inherit: Same as input
  Out1 : Outport  VectorParamsAs1DForOutWhenUnconnected=off
  wires:
  DummyGain/1 -> Out1/1
  In1/1 -> DummyGain/1

== system ASM_Traffic_MultiCore/Drivetrain/Interface_In/ModelSignals/Pos_AccPedal[%]_ ==
  In1 : Inport
  DummyGain : Gain  SaturateOnIntegerOverflow=on  OutDataTypeStr=Inherit: Same as input  ParamDataTypeStr=Inherit: Same as input
  Out1 : Outport  VectorParamsAs1DForOutWhenUnconnected=off
  wires:
  DummyGain/1 -> Out1/1
  In1/1 -> DummyGain/1

== system ASM_Traffic_MultiCore/Drivetrain/Interface_In/ModelSignals/Pos_ClutchPedal[%]_ ==
  In1 : Inport
  DummyGain : Gain  SaturateOnIntegerOverflow=on  OutDataTypeStr=Inherit: Same as input  ParamDataTypeStr=Inherit: Same as input
  Out1 : Outport  VectorParamsAs1DForOutWhenUnconnected=off
  wires:
  In1/1 -> DummyGain/1
  DummyGain/1 -> Out1/1

== system ASM_Traffic_MultiCore/Drivetrain/Interface_In/ModelSignals/Reset_States[0|1]_ ==
  In1 : Inport
  DummyGain : Gain  SaturateOnIntegerOverflow=on  OutDataTypeStr=Inherit: Same as input  ParamDataTypeStr=Inherit: Same as input
  Out1 : Outport  VectorParamsAs1DForOutWhenUnconnected=off
  wires:
  In1/1 -> DummyGain/1
  DummyGain/1 -> Out1/1

== system ASM_Traffic_MultiCore/Drivetrain/Interface_In/ModelSignals/SelectorLever[-3T|-2P|-1R|0N|1D]_ ==
  In1 : Inport
  DummyGain : Gain  SaturateOnIntegerOverflow=on  OutDataTypeStr=Inherit: Same as input  ParamDataTypeStr=Inherit: Same as input
  Out1 : Outport  VectorParamsAs1DForOutWhenUnconnected=off
  wires:
  DummyGain/1 -> Out1/1
  In1/1 -> DummyGain/1

== system ASM_Traffic_MultiCore/Drivetrain/Interface_In/ModelSignals/State_Engine[0|1|2|3|4]_ ==
  In1 : Inport
  DummyGain : Gain  SaturateOnIntegerOverflow=on  OutDataTypeStr=Inherit: Same as input  ParamDataTypeStr=Inherit: Same as input
  Out1 : Outport  VectorParamsAs1DForOutWhenUnconnected=off
  wires:
  DummyGain/1 -> Out1/1
  In1/1 -> DummyGain/1

== system ASM_Traffic_MultiCore/Drivetrain/Interface_In/ModelSignals/State_StartStop[1Off|2NotReady|3Ready|4EngStopped]_ ==
  In1 : Inport
  DummyGain : Gain  SaturateOnIntegerOverflow=on  OutDataTypeStr=Inherit: Same as input  ParamDataTypeStr=Inherit: Same as input
  Out1 : Outport  VectorParamsAs1DForOutWhenUnconnected=off
  wires:
  DummyGain/1 -> Out1/1
  In1/1 -> DummyGain/1

== system ASM_Traffic_MultiCore/Drivetrain/Interface_In/ModelSignals/Sw_ModelDeskPlottingInterface[0Disabled|1Enabled]_ ==
  In1 : Inport
  Gain : Gain
  Out1 : Outport
  wires:
  Gain/1 -> Out1/1
  In1/1 -> Gain/1

== system ASM_Traffic_MultiCore/Drivetrain/Interface_In/ModelSignals/Sw_ModelPortBlocks[0Disabled|1Enabled]_ ==
  In1 : Inport
  Gain : Gain
  Out1 : Outport
  wires:
  Gain/1 -> Out1/1
  In1/1 -> Gain/1

== system ASM_Traffic_MultiCore/Drivetrain/Interface_In/ModelSignals/Sw_Starter[0|1]_ ==
  In1 : Inport
  DummyGain : Gain  SaturateOnIntegerOverflow=on  OutDataTypeStr=Inherit: Same as input  ParamDataTypeStr=Inherit: Same as input
  Out1 : Outport  VectorParamsAs1DForOutWhenUnconnected=off
  wires:
  In1/1 -> DummyGain/1
  DummyGain/1 -> Out1/1

== system ASM_Traffic_MultiCore/Drivetrain/Interface_In/ModelSignals/Sw_Testbench[0Off|1On]_ ==
  In1 : Inport
  DummyGain : Gain  SaturateOnIntegerOverflow=on  OutDataTypeStr=Inherit: Same as input  ParamDataTypeStr=Inherit: Same as input
  Out1 : Outport  VectorParamsAs1DForOutWhenUnconnected=off
  wires:
  In1/1 -> DummyGain/1
  DummyGain/1 -> Out1/1

== system ASM_Traffic_MultiCore/Drivetrain/Interface_In/ModelSignals/Sw_TipShift[-1Down|0Off|1Up]_ ==
  In1 : Inport
  DummyGain : Gain  SaturateOnIntegerOverflow=on  OutDataTypeStr=Inherit: Same as input  ParamDataTypeStr=Inherit: Same as input
  Out1 : Outport  VectorParamsAs1DForOutWhenUnconnected=off
  wires:
  DummyGain/1 -> Out1/1
  In1/1 -> DummyGain/1

== system ASM_Traffic_MultiCore/Drivetrain/Interface_In/ModelSignals/Trq_MeanEff_Engine[Nm]_ ==
  In1 : Inport
  DummyGain : Gain  SaturateOnIntegerOverflow=on  OutDataTypeStr=Inherit: Same as input  ParamDataTypeStr=Inherit: Same as input
  Out1 : Outport  VectorParamsAs1DForOutWhenUnconnected=off
  wires:
  In1/1 -> DummyGain/1
  DummyGain/1 -> Out1/1

== system ASM_Traffic_MultiCore/Drivetrain/Interface_In/ModelSignals/Type_Engine_1[0Unkown|1Other|2Otto|3Diesel|4Electric]_ ==
  In1 : Inport
  DummyGain : Gain  SaturateOnIntegerOverflow=on  OutDataTypeStr=Inherit: Same as input  ParamDataTypeStr=Inherit: Same as input
  Out1 : Outport  VectorParamsAs1DForOutWhenUnconnected=off
  wires:
  DummyGain/1 -> Out1/1
  In1/1 -> DummyGain/1

== system ASM_Traffic_MultiCore/Drivetrain/Interface_In/ModelSignals/n_Engine_Set[rpm]_ ==
  In1 : Inport
  DummyGain : Gain  SaturateOnIntegerOverflow=on  OutDataTypeStr=Inherit: Same as input  ParamDataTypeStr=Inherit: Same as input
  Out1 : Outport  VectorParamsAs1DForOutWhenUnconnected=off
  wires:
  In1/1 -> DummyGain/1
  DummyGain/1 -> Out1/1

== system ASM_Traffic_MultiCore/Drivetrain/Interface_In/ModelSignals/omega_Wheel[FL;FR;RL;RR][rad|s]_ ==
  In1 : Inport
  DummyGain : Gain  SaturateOnIntegerOverflow=on  OutDataTypeStr=Inherit: Same as input  ParamDataTypeStr=Inherit: Same as input
  Out1 : Outport  VectorParamsAs1DForOutWhenUnconnected=off
  wires:
  In1/1 -> DummyGain/1
  DummyGain/1 -> Out1/1

== system ASM_Traffic_MultiCore/Drivetrain/Interface_Out/Animation/Gear[]_ ==
  In1 : Inport
  Gain : Gain  SaturateOnIntegerOverflow=on  OutDataTypeStr=Inherit: Same as input  ParamDataTypeStr=Inherit: Same as input
  Out1 : Outport  VectorParamsAs1DForOutWhenUnconnected=off
  wires:
  In1/1 -> Gain/1
  Gain/1 -> Out1/1

== system ASM_Traffic_MultiCore/Drivetrain/Interface_Out/Animation/n_Engine[rpm]_ ==
  In1 : Inport
  Gain : Gain  SaturateOnIntegerOverflow=on  OutDataTypeStr=Inherit: Same as input  ParamDataTypeStr=Inherit: Same as input
  Out1 : Outport  VectorParamsAs1DForOutWhenUnconnected=off
  wires:
  In1/1 -> Gain/1
  Gain/1 -> Out1/1

== system ASM_Traffic_MultiCore/Drivetrain/Interface_Out/Control_ModelSignals/Ctrl_Parking_Pawl[0|1]_ ==
  In1 : Inport
  DummyGain : Gain  SaturateOnIntegerOverflow=on  OutDataTypeStr=Inherit: Same as input  ParamDataTypeStr=Inherit: Same as input
  Out1 : Outport  VectorParamsAs1DForOutWhenUnconnected=off
  wires:
  DummyGain/1 -> Out1/1
  In1/1 -> DummyGain/1

== system ASM_Traffic_MultiCore/Drivetrain/Interface_Out/Control_ModelSignals/Factor_Trq_Engine_Red[%]_ ==
  In1 : Inport
  Gain : Gain  SaturateOnIntegerOverflow=on  OutDataTypeStr=Inherit: Same as input  ParamDataTypeStr=Inherit: Same as input
  Out1 : Outport  VectorParamsAs1DForOutWhenUnconnected=off
  wires:
  In1/1 -> Gain/1
  Gain/1 -> Out1/1

== system ASM_Traffic_MultiCore/Drivetrain/Interface_Out/Plant_ModelSignals/Gear[]_ ==
  In1 : Inport
  Gain : Gain  SaturateOnIntegerOverflow=on  OutDataTypeStr=Inherit: Same as input  ParamDataTypeStr=Inherit: Same as input
  Out1 : Outport  VectorParamsAs1DForOutWhenUnconnected=off
  wires:
  In1/1 -> Gain/1
  Gain/1 -> Out1/1

== system ASM_Traffic_MultiCore/Drivetrain/Interface_Out/Plant_ModelSignals/Mode_Drivetrain[1|2|3|4|5]_ ==
  In1 : Inport
  DummyGain : Gain  SaturateOnIntegerOverflow=on  OutDataTypeStr=Inherit: Same as input  ParamDataTypeStr=Inherit: Same as input
  Out1 : Outport  VectorParamsAs1DForOutWhenUnconnected=off
  wires:
  In1/1 -> DummyGain/1
  DummyGain/1 -> Out1/1

== system ASM_Traffic_MultiCore/Drivetrain/Interface_Out/Plant_ModelSignals/Mode_Transmission[1Manual|2Automatic]_ ==
  In1 : Inport
  DummyGain : Gain  SaturateOnIntegerOverflow=on  OutDataTypeStr=Inherit: Same as input  ParamDataTypeStr=Inherit: Same as input
  Out1 : Outport  VectorParamsAs1DForOutWhenUnconnected=off
  wires:
  DummyGain/1 -> Out1/1
  In1/1 -> DummyGain/1

== system ASM_Traffic_MultiCore/Drivetrain/Interface_Out/Plant_ModelSignals/Sw_CrankShaft_Reset[0Disabled|1Enabled]_ ==
  In1 : Inport
  DummyGain : Gain  SaturateOnIntegerOverflow=on  OutDataTypeStr=Inherit: Same as input  ParamDataTypeStr=Inherit: Same as input
  Out1 : Outport  VectorParamsAs1DForOutWhenUnconnected=off
  wires:
  In1/1 -> DummyGain/1
  DummyGain/1 -> Out1/1

== system ASM_Traffic_MultiCore/Drivetrain/Interface_Out/Plant_ModelSignals/TrqDistri_Front_Rear[0_1]_ ==
  In1 : Inport
  Gain : Gain  SaturateOnIntegerOverflow=on  OutDataTypeStr=Inherit: Same as input  ParamDataTypeStr=Inherit: Same as input
  Out1 : Outport  VectorParamsAs1DForOutWhenUnconnected=off
  wires:
  Gain/1 -> Out1/1
  In1/1 -> Gain/1

== system ASM_Traffic_MultiCore/Drivetrain/Interface_Out/Plant_ModelSignals/Trq_BSG[Nm]_ ==
  In1 : Inport
  DummyGain : Gain  SaturateOnIntegerOverflow=on  OutDataTypeStr=Inherit: Same as input  ParamDataTypeStr=Inherit: Same as input
  Out1 : Outport  VectorParamsAs1DForOutWhenUnconnected=off
  wires:
  In1/1 -> DummyGain/1
  DummyGain/1 -> Out1/1

== system ASM_Traffic_MultiCore/Drivetrain/Interface_Out/Plant_ModelSignals/Trq_Engine_1[Nm]_ ==
  In1 : Inport
  DummyGain : Gain  SaturateOnIntegerOverflow=on  OutDataTypeStr=Inherit: Same as input  ParamDataTypeStr=Inherit: Same as input
  Out1 : Outport  VectorParamsAs1DForOutWhenUnconnected=off
  wires:
  DummyGain/1 -> Out1/1
  In1/1 -> DummyGain/1

== system ASM_Traffic_MultiCore/Drivetrain/Interface_Out/Plant_ModelSignals/Trq_Engine_2[Nm]_ ==
  In1 : Inport
  DummyGain : Gain  SaturateOnIntegerOverflow=on  OutDataTypeStr=Inherit: Same as input  ParamDataTypeStr=Inherit: Same as input
  Out1 : Outport  VectorParamsAs1DForOutWhenUnconnected=off
  wires:
  DummyGain/1 -> Out1/1
  In1/1 -> DummyGain/1

== system ASM_Traffic_MultiCore/Drivetrain/Interface_Out/Plant_ModelSignals/Trq_Out_Front_Diff[Nm]_ ==
  In1 : Inport
  Gain : Gain  SaturateOnIntegerOverflow=on  OutDataTypeStr=Inherit: Same as input  ParamDataTypeStr=Inherit: Same as input
  Out1 : Outport  VectorParamsAs1DForOutWhenUnconnected=off
  wires:
  In1/1 -> Gain/1
  Gain/1 -> Out1/1

== system ASM_Traffic_MultiCore/Drivetrain/Interface_Out/Plant_ModelSignals/Trq_Shaft[FL;FR;RL;RR][Nm]_ ==
  In1 : Inport
  Gain : Gain  SaturateOnIntegerOverflow=on  OutDataTypeStr=Inherit: Same as input  ParamDataTypeStr=Inherit: Same as input
  Out1 : Outport  VectorParamsAs1DForOutWhenUnconnected=off
  wires:
  In1/1 -> Gain/1
  Gain/1 -> Out1/1

== system ASM_Traffic_MultiCore/Drivetrain/Interface_Out/Plant_ModelSignals/Type_Engine_1[0Unkown|1Other|2Otto|3Diesel|4Electric]_ ==
  In1 : Inport
  DummyGain : Gain  SaturateOnIntegerOverflow=on  OutDataTypeStr=Inherit: Same as input  ParamDataTypeStr=Inherit: Same as input
  Out1 : Outport  VectorParamsAs1DForOutWhenUnconnected=off
  wires:
  DummyGain/1 -> Out1/1
  In1/1 -> DummyGain/1

== system ASM_Traffic_MultiCore/Drivetrain/Interface_Out/Plant_ModelSignals/Type_Engine_2[0Unkown|1Other|2Otto|3Diesel|4Electric]_ ==
  In1 : Inport
  DummyGain : Gain  SaturateOnIntegerOverflow=on  OutDataTypeStr=Inherit: Same as input  ParamDataTypeStr=Inherit: Same as input
  Out1 : Outport  VectorParamsAs1DForOutWhenUnconnected=off
  wires:
  DummyGain/1 -> Out1/1
  In1/1 -> DummyGain/1

== system ASM_Traffic_MultiCore/Drivetrain/Interface_Out/Plant_ModelSignals/i_FinalDrive[]_ ==
  In1 : Inport
  Gain : Gain  SaturateOnIntegerOverflow=on  OutDataTypeStr=Inherit: Same as input  ParamDataTypeStr=Inherit: Same as input
  Out1 : Outport  VectorParamsAs1DForOutWhenUnconnected=off
  wires:
  In1/1 -> Gain/1
  Gain/1 -> Out1/1

== system ASM_Traffic_MultiCore/Drivetrain/Interface_Out/Plant_ModelSignals/i_FrontDrive[]_ ==
  In1 : Inport
  Gain : Gain  SaturateOnIntegerOverflow=on  OutDataTypeStr=Inherit: Same as input  ParamDataTypeStr=Inherit: Same as input
  Out1 : Outport  VectorParamsAs1DForOutWhenUnconnected=off
  wires:
  In1/1 -> Gain/1
  Gain/1 -> Out1/1

== system ASM_Traffic_MultiCore/Drivetrain/Interface_Out/Plant_ModelSignals/i_RearDrive[]_ ==
  In1 : Inport
  Gain : Gain  SaturateOnIntegerOverflow=on  OutDataTypeStr=Inherit: Same as input  ParamDataTypeStr=Inherit: Same as input
  Out1 : Outport  VectorParamsAs1DForOutWhenUnconnected=off
  wires:
  In1/1 -> Gain/1
  Gain/1 -> Out1/1

== system ASM_Traffic_MultiCore/Drivetrain/Interface_Out/Plant_ModelSignals/i_unsync_Trm[]_ ==
  In1 : Inport
  Gain : Gain  SaturateOnIntegerOverflow=on  OutDataTypeStr=Inherit: Same as input  ParamDataTypeStr=Inherit: Same as input
  Out1 : Outport  VectorParamsAs1DForOutWhenUnconnected=off
  wires:
  In1/1 -> Gain/1
  Gain/1 -> Out1/1

== system ASM_Traffic_MultiCore/Drivetrain/Interface_Out/Plant_ModelSignals/n_Engine[rpm]_ ==
  In1 : Inport
  Gain : Gain  SaturateOnIntegerOverflow=on  OutDataTypeStr=Inherit: Same as input  ParamDataTypeStr=Inherit: Same as input
  Out1 : Outport  VectorParamsAs1DForOutWhenUnconnected=off
  wires:
  In1/1 -> Gain/1
  Gain/1 -> Out1/1

== system ASM_Traffic_MultiCore/Drivetrain/Interface_Out/Plant_ModelSignals/n_Engine_1[rpm]_ ==
  In1 : Inport
  DummyGain : Gain  SaturateOnIntegerOverflow=on  OutDataTypeStr=Inherit: Same as input  ParamDataTypeStr=Inherit: Same as input
  Out1 : Outport  VectorParamsAs1DForOutWhenUnconnected=off
  wires:
  DummyGain/1 -> Out1/1
  In1/1 -> DummyGain/1

== system ASM_Traffic_MultiCore/Drivetrain/Interface_Out/Plant_ModelSignals/n_Engine_2[rpm]_ ==
  In1 : Inport
  DummyGain : Gain  SaturateOnIntegerOverflow=on  OutDataTypeStr=Inherit: Same as input  ParamDataTypeStr=Inherit: Same as input
  Out1 : Outport  VectorParamsAs1DForOutWhenUnconnected=off
  wires:
  DummyGain/1 -> Out1/1
  In1/1 -> DummyGain/1

== system ASM_Traffic_MultiCore/Drivetrain/Interface_Out/Plant_ModelSignals/omega_Out_Trm[rad|s]_ ==
  In1 : Inport
  Gain : Gain  SaturateOnIntegerOverflow=on  OutDataTypeStr=Inherit: Same as input  ParamDataTypeStr=Inherit: Same as input
  Out1 : Outport  VectorParamsAs1DForOutWhenUnconnected=off
  wires:
  In1/1 -> Gain/1
  Gain/1 -> Out1/1

== system ASM_Traffic_MultiCore/Drivetrain/Plant/Drivetrain/ASMSignalCollector ==
  Interface_In : Inport
  Bus Selector : BusSelector  OutputSignals=ExternalModel.Type_Engine_1[0Unkown|1Other|2Otto|3Diesel|4Electric],ExternalModel.Trq_MeanEff_Engine[Nm]
  BusCreator : BusCreator  Inputs=7
  ASMSignalBus : Outport  VectorParamsAs1DForOutWhenUnconnected=off
  wires:
  [ASMBUS_Drivetrain_FinalDriveAssembly] -> BusCreator/5
  [ASMBUS_Drivetrain_Transmission] -> BusCreator/4
  [ASMBUS_Drivetrain_TestBench] -> BusCreator/3
  [ASMBUS_Drivetrain_Starter] -> BusCreator/2
  [ASMBUS_Drivetrain_Crankshaft] -> BusCreator/1
  BusCreator/1 -> ASMSignalBus/1  "Drivetrain"
  Interface_In/1 -> Bus Selector/1
  Bus Selector/1 -> BusCreator/6  "<Type_Engine_1[0Unkown|1Other|2Otto|3Diesel|4Electric]>"
  Bus Selector/2 -> BusCreator/7  "<Trq_MeanEff_Engine[Nm]>"

== system ASM_Traffic_MultiCore/Drivetrain/Plant/Drivetrain/Crankshaft ==
  Trq_TestBench[Nm] : Inport
  Inertia_External[kgm2] : Inport  Port=2
  Trq_External[Nm] : Inport  Port=3
  CrankAngle_Cyl[deg] : Inport  Port=4
  Trq_Engine[Nm] : Inport  Port=5
  Reset[0|1] : Inport  Port=6
  Trq_Fric_Clutch[Nm] : Inport  Port=7
  omega_In_Trm[rad|s] : Inport  Port=8
  CRANK_SHAFT_RIGID : ASM_VehicleDynamics_lib/Drivetrain/Crankshaft_and_Starter/CRANK_SHAFT_RIGID  Tag=ASM_SUBCOMPONENT  Const_Inertia=MDL.Drivetrain.CrankShaftRigid.Const_Inertia  Map_Trq_Mass_Mod=MDL.Drivetrain.CrankShaftRigid.Map_Trq_Mass_Mod  Sw_Trq_Mass_Mode=MDL.Drivetrain.CrankShaftRigid.Sw_Trq_Mass_Mode  StepSize=SIM.StepSize  ASMProperties=struct('Name','CRANK_SHAFT_RIGID','Version','4.0','Library','ASM_VehicleDynamics_lib')  ASMInstanceName=crank_shaft_rigid  ASMInstanceID=1
  Memory : Memory
  n_Engine[rpm] : Outport  VectorParamsAs1DForOutWhenUnconnected=off
  n_Engine[rad|s] : Outport  Port=2  VectorParamsAs1DForOutWhenUnconnected=off
  tag scope: ASMBUS_Drivetrain_Crankshaft=scoped
  wires:
  Memory/1 -> CRANK_SHAFT_RIGID/8
  Trq_Fric_Clutch[Nm]/1 -> CRANK_SHAFT_RIGID/3
  Trq_TestBench[Nm]/1 -> CRANK_SHAFT_RIGID/6
  Reset[0|1]/1 -> CRANK_SHAFT_RIGID/4
  Inertia_External[kgm2]/1 -> CRANK_SHAFT_RIGID/5
  Trq_External[Nm]/1 -> CRANK_SHAFT_RIGID/1
  omega_In_Trm[rad|s]/1 -> Memory/1
  Trq_Engine[Nm]/1 -> CRANK_SHAFT_RIGID/2
  CrankAngle_Cyl[deg]/1 -> CRANK_SHAFT_RIGID/7
  CRANK_SHAFT_RIGID/3 -> n_Engine[rad|s]/1
  CRANK_SHAFT_RIGID/2 -> n_Engine[rpm]/1
  CRANK_SHAFT_RIGID/1 -> [ASMBUS_Drivetrain_Crankshaft]

== system ASM_Traffic_MultiCore/Drivetrain/Plant/Drivetrain/DisableReset ==
  Reset_States[0|1] : Inport
  Sw_CrankShaft_Reset[0Disabled|1Enabled] : Inport  Port=2
  MultiPortSwitch : MultiPortSwitch  DataPortOrder=Zero-based contiguous  Inputs=2  zeroidx=on
  NO_Reset : Constant  Value=0
  Reset[0|1] : Outport  VectorParamsAs1DForOutWhenUnconnected=off
  wires:
  Reset_States[0|1]/1 -> MultiPortSwitch/3
  NO_Reset/1 -> MultiPortSwitch/2
  Sw_CrankShaft_Reset[0Disabled|1Enabled]/1 -> MultiPortSwitch/1
  MultiPortSwitch/1 -> Reset[0|1]/1

== system ASM_Traffic_MultiCore/Drivetrain/Plant/Drivetrain/External_Loads ==
  Inertia_TestBench[kgm2] : Inport
  Trq_Starter[Nm] : Inport  Port=2
  Inertia_Starter[kgm2] : Inport  Port=3
  UserInterface : Inport  Port=4
  Add : Sum
  Bus Selector3 : BusSelector  OutputSignals=Const_LoadTorque[Nm],Sw_LoadTorque[0Clutch|1Constant]
  Switch : Switch  Criteria=u2 ~= 0  SaturateOnIntegerOverflow=off  InputSameDT=off
  Inertia_External[kgm2] : Outport  VectorParamsAs1DForOutWhenUnconnected=off
  Trq_External[Nm] : Outport  Port=2  VectorParamsAs1DForOutWhenUnconnected=off
  wires:
  Inertia_Starter[kgm2]/1 -> Add/1
  Switch/1 -> Trq_External[Nm]/1
  Add/1 -> Inertia_External[kgm2]/1
  Inertia_TestBench[kgm2]/1 -> Add/2
  UserInterface/1 -> Bus Selector3/1
  Trq_Starter[Nm]/1 -> Switch/3
  Bus Selector3/1 -> Switch/1  "<Const_LoadTorque[Nm]>"
  Bus Selector3/2 -> Switch/2  "<Sw_LoadTorque[0Clutch|1Constant]>"
